simulink model "simulate_gofa_2023"  (R2023a)
settings: Solver=FixedStepAuto  StartTime=0.0  StopTime=100  RelTol=1e-3
undefined symbols (not defined in the file or in its folder): X, Y, Z
libraries: sm_lib x126, nesl_utility x14
(part 3 of 3)

== system simulate_gofa_2023/GOFA robot/link_6 ==
  ReferenceFrame : sm_lib/Frames and Transforms/Reference Frame
  Visual : sm_lib/Body Elements/File Solid  ExtGeomFileName=link_6.stl  UnitType=Custom  ExtGeomFileUnits=m  StepReaderType=HEX  ExportConvexHullGeometry=off  InertiaType=Custom  BasedOnType=DensityFromFile  Density=1000  DensityUnits=kg/m^3  Mass=0  MassUnits=kg  CenterOfMass=[0, 0, 0]  CenterOfMassUnits=m  MomentsOfInertia=[0, 0, 0]  MomentsOfInertiaUnits=kg*m^2  ProductsOfInertia=[0, 0, 0]  ProductsOfInertiaUnits=kg*m^2  GraphicType=FromGeometry  MarkerShape=Sphere  MarkerSize=10  GraphicVisPropType=SimpleVisualProperties  GraphicDiffuseColor=[0.8392157, 0.8352941, 0.7921569000000001]  GraphicOpacity=1  GraphicSpecularColor=[0.5 0.5 0.5 1.0]  GraphicAmbientColor=[0.15 0.15 0.15 1.0]  GraphicEmissiveColor=[0.0 0.0 0.0 1.0]  GraphicShininess=75  DoExposeReferenceFrame=on  SerializedFrames=<Frames/>
  VisualOriginTransform : sm_lib/Frames and Transforms/Rigid Transform  RotationMethod=RotationSequence  FollAlignAxisA=+X  BaseAlignAxisA=+Y  FollAlignAxisB=+Y  BaseAlignAxisB=+Z  RotationStandardAxis=+Z  RotationAngle=0  RotationAngleUnits=deg  RotationArbitraryAxis=[0 0 1]  RotationSequenceAxes=BaseAxes  RotationSequence=XYZ  RotationSequenceAngles=[0, 0, 0]  RotationSequenceAnglesUnits=rad  RotationMatrix=[1 0 0;0 1 0;0 0 1]  Quaternion=[1 0 0 0]  TranslationMethod=Cartesian  TranslationCartesianOffset=[0, 0, 0]  TranslationCartesianOffsetUnits=m  TranslationStandardAxis=+Z  TranslationStandardOffset=0  TranslationStandardOffsetUnits=m  TranslationROffset=0  TranslationROffsetUnits=m  TranslationThetaOffset=0  TranslationThetaOffsetUnits=deg  TranslationZOffset=0  TranslationZOffsetUnits=m
  joint_6_AxisInvTransform : sm_lib/Frames and Transforms/Rigid Transform  RotationMethod=ArbitraryAxis  FollAlignAxisA=+X  BaseAlignAxisA=+Y  FollAlignAxisB=+Y  BaseAlignAxisB=+Z  RotationStandardAxis=+Z  RotationAngle=1.570796326794897  RotationAngleUnits=rad  RotationArbitraryAxis=[-0, 1, 0]  RotationSequenceAxes=FollowerAxes  RotationSequence=XYX  RotationSequenceAngles=[0 0 0]  RotationSequenceAnglesUnits=deg  RotationMatrix=[1 0 0;0 1 0;0 0 1]  Quaternion=[1 0 0 0]  TranslationMethod=Cartesian  TranslationCartesianOffset=[0, 0, 0]  TranslationCartesianOffsetUnits=m  TranslationStandardAxis=+Z  TranslationStandardOffset=0  TranslationStandardOffsetUnits=m  TranslationROffset=0  TranslationROffsetUnits=m  TranslationThetaOffset=0  TranslationThetaOffsetUnits=deg  TranslationZOffset=0  TranslationZOffsetUnits=m
  joint_6_flange_OriginTransform : sm_lib/Frames and Transforms/Rigid Transform  RotationMethod=RotationSequence  FollAlignAxisA=+X  BaseAlignAxisA=+Y  FollAlignAxisB=+Y  BaseAlignAxisB=+Z  RotationStandardAxis=+Z  RotationAngle=0  RotationAngleUnits=deg  RotationArbitraryAxis=[0 0 1]  RotationSequenceAxes=BaseAxes  RotationSequence=XYZ  RotationSequenceAngles=[0, 0, 0]  RotationSequenceAnglesUnits=rad  RotationMatrix=[1 0 0;0 1 0;0 0 1]  Quaternion=[1 0 0 0]  TranslationMethod=Cartesian  TranslationCartesianOffset=[0, 0, 0]  TranslationCartesianOffsetUnits=m  TranslationStandardAxis=+Z  TranslationStandardOffset=0  TranslationStandardOffsetUnits=m  TranslationROffset=0  TranslationROffsetUnits=m  TranslationThetaOffset=0  TranslationThetaOffsetUnits=deg  TranslationZOffset=0  TranslationZOffsetUnits=m
  F : PMIOPort  Side=Left
  F1 : PMIOPort  Port=2  Side=Right
  connections:
  ReferenceFrame/RConn1 -- VisualOriginTransform/LConn1 -- joint_6_AxisInvTransform/LConn1 -- joint_6_flange_OriginTransform/LConn1
  Visual/RConn1 -- VisualOriginTransform/RConn1
  joint_6_AxisInvTransform/RConn1 -- F/RConn1
  joint_6_flange_OriginTransform/RConn1 -- F1/RConn1

== system simulate_gofa_2023/GOFA robot/tool0 ==
  ReferenceFrame : sm_lib/Frames and Transforms/Reference Frame
  F : PMIOPort  Side=Left
  connections:
  ReferenceFrame/RConn1 -- F/RConn1

== matlab function simulate_gofa_2023/GOFA ROBOT KINEMATIC ==
  data: x output; t1 input; y output; t2 input; t3 input; t4 input; t5 input; t6 input; z output; R output
function [x,y,z,R] = fcn(t1,t2,t3,t4,t5,t6)

% Constant params
% d3= 0.15;
% a2 = 0.4318;
% a3 = 0.0203;
% d4 = 0.4318;
% d5 = 0.1;

% end effector position
x = (646333333153388974303668854092654500447200796230458690753650903093*sin((180*t1)/pi))/3291009114642412084309938365114701009965471731267159726697218048000 + (1641179897212867899457543764218157*cos((180*t4)/pi)*((16210310927856405661316834439721*sin((180*t1)/pi))/20282409603651670423947251286016 - (4035888341267763*cos((180*t3)/pi)*((4035888341267763*cos((180*t2)/pi - 90)*sin((180*t1)/pi))/9007199254740992 - sin((180*t2)/pi - 90)*cos((180*t1)/pi)))/9007199254740992 + (4035888341267763*sin((180*t3)/pi)*(cos((180*t2)/pi - 90)*cos((180*t1)/pi) + (4035888341267763*sin((180*t2)/pi - 90)*sin((180*t1)/pi))/9007199254740992))/9007199254740992))/40564819207303340847894502572032000 + (11*cos((180*t3)/pi)*(cos((180*t2)/pi - 90)*cos((180*t1)/pi) + (4035888341267763*sin((180*t2)/pi - 90)*sin((180*t1)/pi))/9007199254740992))/100 + (160146485358502555991456785001454542799219708017911*cos((180*t3)/pi)*((4035888341267763*cos((180*t2)/pi - 90)*sin((180*t1)/pi))/9007199254740992 - sin((180*t2)/pi - 90)*cos((180*t1)/pi)))/365375409332725729550921208179070754913983135744000 - (160146485358502555991456785001454542799219708017911*sin((180*t3)/pi)*(cos((180*t2)/pi - 90)*cos((180*t1)/pi) + (4035888341267763*sin((180*t2)/pi - 90)*sin((180*t1)/pi))/9007199254740992))/365375409332725729550921208179070754913983135744000 + (11*sin((180*t3)/pi)*((4035888341267763*cos((180*t2)/pi - 90)*sin((180*t1)/pi))/9007199254740992 - sin((180*t2)/pi - 90)*cos((180*t1)/pi)))/100 + (2*cos((180*t5)/pi)*(sin((180*t4)/pi)*((16210310927856405661316834439721*sin((180*t1)/pi))/20282409603651670423947251286016 - (4035888341267763*cos((180*t3)/pi)*((4035888341267763*cos((180*t2)/pi - 90)*sin((180*t1)/pi))/9007199254740992 - sin((180*t2)/pi - 90)*cos((180*t1)/pi)))/9007199254740992 + (4035888341267763*sin((180*t3)/pi)*(cos((180*t2)/pi - 90)*cos((180*t1)/pi) + (4035888341267763*sin((180*t2)/pi - 90)*sin((180*t1)/pi))/9007199254740992))/9007199254740992) + cos((180*t4)/pi)*(cos((180*t3)/pi)*(cos((180*t2)/pi - 90)*cos((180*t1)/pi) + (4035888341267763*sin((180*t2)/pi - 90)*sin((180*t1)/pi))/9007199254740992) + sin((180*t3)/pi)*((4035888341267763*cos((180*t2)/pi - 90)*sin((180*t1)/pi))/9007199254740992 - sin((180*t2)/pi - 90)*cos((180*t1)/pi)))))/25 - (1641179897212867899457543764218157*sin((180*t4)/pi)*(cos((180*t3)/pi)*(cos((180*t2)/pi - 90)*cos((180*t1)/pi) + (4035888341267763*sin((180*t2)/pi - 90)*sin((180*t1)/pi))/9007199254740992) + sin((180*t3)/pi)*((4035888341267763*cos((180*t2)/pi - 90)*sin((180*t1)/pi))/9007199254740992 - sin((180*t2)/pi - 90)*cos((180*t1)/pi))))/40564819207303340847894502572032000 - (406646507147255839*sin((180*t5)/pi)*(sin((180*t4)/pi)*((16210310927856405661316834439721*sin((180*t1)/pi))/20282409603651670423947251286016 - (4035888341267763*cos((180*t3)/pi)*((4035888341267763*cos((180*t2)/pi - 90)*sin((180*t1)/pi))/9007199254740992 - sin((180*t2)/pi - 90)*cos((180*t1)/pi)))/9007199254740992 + (4035888341267763*sin((180*t3)/pi)*(cos((180*t2)/pi - 90)*cos((180*t1)/pi) + (4035888341267763*sin((180*t2)/pi - 90)*sin((180*t1)/pi))/9007199254740992))/9007199254740992) + cos((180*t4)/pi)*(cos((180*t3)/pi)*(cos((180*t2)/pi - 90)*cos((180*t1)/pi) + (4035888341267763*sin((180*t2)/pi - 90)*sin((180*t1)/pi))/9007199254740992) + sin((180*t3)/pi)*((4035888341267763*cos((180*t2)/pi - 90)*sin((180*t1)/pi))/9007199254740992 - sin((180*t2)/pi - 90)*cos((180*t1)/pi)))))/4503599627370496000 + (11*cos((180*t2)/pi - 90)*cos((180*t1)/pi))/25 + (406646507147255839*cos((180*t5)/pi)*((65423004882061081215650621571388430732944014123*sin((180*t1)/pi))/182687704666362864775460604089535377456991567872 - (4035888341267763*cos((180*t4)/pi)*((16210310927856405661316834439721*sin((180*t1)/pi))/20282409603651670423947251286016 - (4035888341267763*cos((180*t3)/pi)*((4035888341267763*cos((180*t2)/pi - 90)*sin((180*t1)/pi))/9007199254740992 - sin((180*t2)/pi - 90)*cos((180*t1)/pi)))/9007199254740992 + (4035888341267763*sin((180*t3)/pi)*(cos((180*t2)/pi - 90)*cos((180*t1)/pi) + (4035888341267763*sin((180*t2)/pi - 90)*sin((180*t1)/pi))/9007199254740992))/9007199254740992))/9007199254740992 + (16210310927856405661316834439721*cos((180*t3)/pi)*((4035888341267763*cos((180*t2)/pi - 90)*sin((180*t1)/pi))/9007199254740992 - sin((180*t2)/pi - 90)*cos((180*t1)/pi)))/20282409603651670423947251286016 - (16210310927856405661316834439721*sin((180*t3)/pi)*(cos((180*t2)/pi - 90)*cos((180*t1)/pi) + (4035888341267763*sin((180*t2)/pi - 90)*sin((180*t1)/pi))/9007199254740992))/20282409603651670423947251286016 + (4035888341267763*sin((180*t4)/pi)*(cos((180*t3)/pi)*(cos((180*t2)/pi - 90)*cos((180*t1)/pi) + (4035888341267763*sin((180*t2)/pi - 90)*sin((180*t1)/pi))/9007199254740992) + sin((180*t3)/pi)*((4035888341267763*cos((180*t2)/pi - 90)*sin((180*t1)/pi))/9007199254740992 - sin((180*t2)/pi - 90)*cos((180*t1)/pi))))/9007199254740992))/4503599627370496000 + (44394771753945393*sin((180*t2)/pi - 90)*sin((180*t1)/pi))/225179981368524800 + (2*sin((180*t5)/pi)*((65423004882061081215650621571388430732944014123*sin((180*t1)/pi))/182687704666362864775460604089535377456991567872 - (4035888341267763*cos((180*t4)/pi)*((16210310927856405661316834439721*sin((180*t1)/pi))/20282409603651670423947251286016 - (4035888341267763*cos((180*t3)/pi)*((4035888341267763*cos((180*t2)/pi - 90)*sin((180*t1)/pi))/9007199254740992 - sin((180*t2)/pi - 90)*cos((180*t1)/pi)))/9007199254740992 + (4035888341267763*sin((180*t3)/pi)*(cos((180*t2)/pi - 90)*cos((180*t1)/pi) + (4035888341267763*sin((180*t2)/pi - 90)*sin((180*t1)/pi))/9007199254740992))/9007199254740992))/9007199254740992 + (16210310927856405661316834439721*cos((180*t3)/pi)*((4035888341267763*cos((180*t2)/pi - 90)*sin((180*t1)/pi))/9007199254740992 - sin((180*t2)/pi - 90)*cos((180*t1)/pi)))/20282409603651670423947251286016 - (16210310927856405661316834439721*sin((180*t3)/pi)*(cos((180*t2)/pi - 90)*cos((180*t1)/pi) + (4035888341267763*sin((180*t2)/pi - 90)*sin((180*t1)/pi))/9007199254740992))/20282409603651670423947251286016 + (4035888341267763*sin((180*t4)/pi)*(cos((180*t3)/pi)*(cos((180*t2)/pi - 90)*cos((180*t1)/pi) + (4035888341267763*sin((180*t2)/pi - 90)*sin((180*t1)/pi))/9007199254740992) + sin((180*t3)/pi)*((4035888341267763*cos((180*t2)/pi - 90)*sin((180*t1)/pi))/9007199254740992 - sin((180*t2)/pi - 90)*cos((180*t1)/pi))))/9007199254740992))/25;

y = (1641179897212867899457543764218157*cos((180*t4)/pi)*((4035888341267763*cos((180*t3)/pi)*((4035888341267763*cos((180*t2)/pi - 90)*cos((180*t1)/pi))/9007199254740992 + sin((180*t2)/pi - 90)*sin((180*t1)/pi)))/9007199254740992 - (16210310927856405661316834439721*cos((180*t1)/pi))/20282409603651670423947251286016 + (4035888341267763*sin((180*t3)/pi)*(cos((180*t2)/pi - 90)*sin((180*t1)/pi) - (4035888341267763*sin((180*t2)/pi - 90)*cos((180*t1)/pi))/9007199254740992))/9007199254740992))/40564819207303340847894502572032000 - (646333333153388974303668854092654500447200796230458690753650903093*cos((180*t1)/pi))/3291009114642412084309938365114701009965471731267159726697218048000 + (11*cos((180*t3)/pi)*(cos((180*t2)/pi - 90)*sin((180*t1)/pi) - (4035888341267763*sin((180*t2)/pi - 90)*cos((180*t1)/pi))/9007199254740992))/100 - (160146485358502555991456785001454542799219708017911*cos((180*t3)/pi)*((4035888341267763*cos((180*t2)/pi - 90)*cos((180*t1)/pi))/9007199254740992 + sin((180*t2)/pi - 90)*sin((180*t1)/pi)))/365375409332725729550921208179070754913983135744000 + (2*cos((180*t5)/pi)*(sin((180*t4)/pi)*((4035888341267763*cos((180*t3)/pi)*((4035888341267763*cos((180*t2)/pi - 90)*cos((180*t1)/pi))/9007199254740992 + sin((180*t2)/pi - 90)*sin((180*t1)/pi)))/9007199254740992 - (16210310927856405661316834439721*cos((180*t1)/pi))/20282409603651670423947251286016 + (4035888341267763*sin((180*t3)/pi)*(cos((180*t2)/pi - 90)*sin((180*t1)/pi) - (4035888341267763*sin((180*t2)/pi - 90)*cos((180*t1)/pi))/9007199254740992))/9007199254740992) + cos((180*t4)/pi)*(cos((180*t3)/pi)*(cos((180*t2)/pi - 90)*sin((180*t1)/pi) - (4035888341267763*sin((180*t2)/pi - 90)*cos((180*t1)/pi))/9007199254740992) - sin((180*t3)/pi)*((4035888341267763*cos((180*t2)/pi - 90)*cos((180*t1)/pi))/9007199254740992 + sin((180*t2)/pi - 90)*sin((180*t1)/pi)))))/25 - (160146485358502555991456785001454542799219708017911*sin((180*t3)/pi)*(cos((180*t2)/pi - 90)*sin((180*t1)/pi) - (4035888341267763*sin((180*t2)/pi - 90)*cos((180*t1)/pi))/9007199254740992))/365375409332725729550921208179070754913983135744000 - (11*sin((180*t3)/pi)*((4035888341267763*cos((180*t2)/pi - 90)*cos((180*t1)/pi))/9007199254740992 + sin((180*t2)/pi - 90)*sin((180*t1)/pi)))/100 - (406646507147255839*sin((180*t5)/pi)*(sin((180*t4)/pi)*((4035888341267763*cos((180*t3)/pi)*((4035888341267763*cos((180*t2)/pi - 90)*cos((180*t1)/pi))/9007199254740992 + sin((180*t2)/pi - 90)*sin((180*t1)/pi)))/9007199254740992 - (16210310927856405661316834439721*cos((180*t1)/pi))/20282409603651670423947251286016 + (4035888341267763*sin((180*t3)/pi)*(cos((180*t2)/pi - 90)*sin((180*t1)/pi) - (4035888341267763*sin((180*t2)/pi - 90)*cos((180*t1)/pi))/9007199254740992))/9007199254740992) + cos((180*t4)/pi)*(cos((180*t3)/pi)*(cos((180*t2)/pi - 90)*sin((180*t1)/pi) - (4035888341267763*sin((180*t2)/pi - 90)*cos((180*t1)/pi))/9007199254740992) - sin((180*t3)/pi)*((4035888341267763*cos((180*t2)/pi - 90)*cos((180*t1)/pi))/9007199254740992 + sin((180*t2)/pi - 90)*sin((180*t1)/pi)))))/4503599627370496000 - (1641179897212867899457543764218157*sin((180*t4)/pi)*(cos((180*t3)/pi)*(cos((180*t2)/pi - 90)*sin((180*t1)/pi) - (4035888341267763*sin((180*t2)/pi - 90)*cos((180*t1)/pi))/9007199254740992) - sin((180*t3)/pi)*((4035888341267763*cos((180*t2)/pi - 90)*cos((180*t1)/pi))/9007199254740992 + sin((180*t2)/pi - 90)*sin((180*t1)/pi))))/40564819207303340847894502572032000 - (406646507147255839*cos((180*t5)/pi)*((65423004882061081215650621571388430732944014123*cos((180*t1)/pi))/182687704666362864775460604089535377456991567872 + (4035888341267763*cos((180*t4)/pi)*((4035888341267763*cos((180*t3)/pi)*((4035888341267763*cos((180*t2)/pi - 90)*cos((180*t1)/pi))/9007199254740992 + sin((180*t2)/pi - 90)*sin((180*t1)/pi)))/9007199254740992 - (16210310927856405661316834439721*cos((180*t1)/pi))/20282409603651670423947251286016 + (4035888341267763*sin((180*t3)/pi)*(cos((180*t2)/pi - 90)*sin((180*t1)/pi) - (4035888341267763*sin((180*t2)/pi - 90)*cos((180*t1)/pi))/9007199254740992))/9007199254740992))/9007199254740992 + (16210310927856405661316834439721*cos((180*t3)/pi)*((4035888341267763*cos((180*t2)/pi - 90)*cos((180*t1)/pi))/9007199254740992 + sin((180*t2)/pi - 90)*sin((180*t1)/pi)))/20282409603651670423947251286016 + (16210310927856405661316834439721*sin((180*t3)/pi)*(cos((180*t2)/pi - 90)*sin((180*t1)/pi) - (4035888341267763*sin((180*t2)/pi - 90)*cos((180*t1)/pi))/9007199254740992))/20282409603651670423947251286016 - (4035888341267763*sin((180*t4)/pi)*(cos((180*t3)/pi)*(cos((180*t2)/pi - 90)*sin((180*t1)/pi) - (4035888341267763*sin((180*t2)/pi - 90)*cos((180*t1)/pi))/9007199254740992) - sin((180*t3)/pi)*((4035888341267763*cos((180*t2)/pi - 90)*cos((180*t1)/pi))/9007199254740992 + sin((180*t2)/pi - 90)*sin((180*t1)/pi))))/9007199254740992))/4503599627370496000 - (2*sin((180*t5)/pi)*((65423004882061081215650621571388430732944014123*cos((180*t1)/pi))/182687704666362864775460604089535377456991567872 + (4035888341267763*cos((180*t4)/pi)*((4035888341267763*cos((180*t3)/pi)*((4035888341267763*cos((180*t2)/pi - 90)*cos((180*t1)/pi))/9007199254740992 + sin((180*t2)/pi - 90)*sin((180*t1)/pi)))/9007199254740992 - (16210310927856405661316834439721*cos((180*t1)/pi))/20282409603651670423947251286016 + (4035888341267763*sin((180*t3)/pi)*(cos((180*t2)/pi - 90)*sin((180*t1)/pi) - (4035888341267763*sin((180*t2)/pi - 90)*cos((180*t1)/pi))/9007199254740992))/9007199254740992))/9007199254740992 + (16210310927856405661316834439721*cos((180*t3)/pi)*((4035888341267763*cos((180*t2)/pi - 90)*cos((180*t1)/pi))/9007199254740992 + sin((180*t2)/pi - 90)*sin((180*t1)/pi)))/20282409603651670423947251286016 + (16210310927856405661316834439721*sin((180*t3)/pi)*(cos((180*t2)/pi - 90)*sin((180*t1)/pi) - (4035888341267763*sin((180*t2)/pi - 90)*cos((180*t1)/pi))/9007199254740992))/20282409603651670423947251286016 - (4035888341267763*sin((180*t4)/pi)*(cos((180*t3)/pi)*(cos((180*t2)/pi - 90)*sin((180*t1)/pi) - (4035888341267763*sin((180*t2)/pi - 90)*cos((180*t1)/pi))/9007199254740992) - sin((180*t3)/pi)*((4035888341267763*cos((180*t2)/pi - 90)*cos((180*t1)/pi))/9007199254740992 + sin((180*t2)/pi - 90)*sin((180*t1)/pi))))/9007199254740992))/25 + (11*cos((180*t2)/pi - 90)*sin((180*t1)/pi))/25 - (44394771753945393*sin((180*t2)/pi - 90)*cos((180*t1)/pi))/225179981368524800;

z = (6607723493088169202780712778710231504027345426423*sin((180*t2)/pi + (180*t3)/pi - 90)*sin((180*t4)/pi))/182687704666362864775460604089535377456991567872000 - (644782266365784279295696367608494311447688133775286220162272389429*cos((180*t2)/pi + (180*t3)/pi - 90))/1645504557321206042154969182557350504982735865633579863348609024000 - (44288233451681329*sin((180*t2)/pi + (180*t3)/pi - 90))/450359962737049600 - cos((180*t5)/pi)*((26540192218155861146320042886836656302738191977718887318238341941*cos((180*t2)/pi + (180*t3)/pi - 90))/411376139330301510538742295639337626245683966408394965837152256000 + (406646507147255839*cos((180*t4)/pi)*((65580384287964744588230398513542208987583003691*cos((180*t2)/pi + (180*t3)/pi - 90))/365375409332725729550921208179070754913983135744 + 65580384287964744588230398513542208987583003691/365375409332725729550921208179070754913983135744))/4503599627370496000 + (6607723493088169202780712778710231504027345426423*sin((180*t2)/pi + (180*t3)/pi - 90)*sin((180*t4)/pi))/182687704666362864775460604089535377456991567872000 - 26668034208075640036217710933510508340280645669893133127658301749/1645504557321206042154969182557350504982735865633579863348609024000) - sin((180*t5)/pi)*((406646507147255839*sin((180*t4)/pi)*((16249305912998692073837066972457*cos((180*t2)/pi + (180*t3)/pi - 90))/40564819207303340847894502572032 + 16249305912998692073837066972457/40564819207303340847894502572032))/4503599627370496000 - (1637241403713496971793000278411821*sin((180*t2)/pi + (180*t3)/pi - 90)*cos((180*t4)/pi))/20282409603651670423947251286016000) - (44288233451681329*sin((180*t2)/pi - 90))/112589990684262400 + cos((180*t5)/pi)*((2*sin((180*t4)/pi)*((16249305912998692073837066972457*cos((180*t2)/pi + (180*t3)/pi - 90))/40564819207303340847894502572032 + 16249305912998692073837066972457/40564819207303340847894502572032))/25 - (4026203041061939*sin((180*t2)/pi + (180*t3)/pi - 90)*cos((180*t4)/pi))/56294995342131200) - sin((180*t5)/pi)*((65266003154295042533483952795954524799922879019*cos((180*t2)/pi + (180*t3)/pi - 90))/1141798154164767904846628775559596109106197299200 + (2*cos((180*t4)/pi)*((65580384287964744588230398513542208987583003691*cos((180*t2)/pi + (180*t3)/pi - 90))/365375409332725729550921208179070754913983135744 + 65580384287964744588230398513542208987583003691/365375409332725729550921208179070754913983135744))/25 + (16249305912998692073837066972457*sin((180*t2)/pi + (180*t3)/pi - 90)*sin((180*t4)/pi))/507060240091291760598681282150400 - 65580384287964744588230398513542208987583003691/4567192616659071619386515102238384436424789196800) + cos((180*t4)/pi)*((26668034208075640036217710933510508340280645669893133127658301749*cos((180*t2)/pi + (180*t3)/pi - 90))/1645504557321206042154969182557350504982735865633579863348609024000 + 26668034208075640036217710933510508340280645669893133127658301749/1645504557321206042154969182557350504982735865633579863348609024000) + 2392122961896179351406805570435440567063495989399766582953892685621/6582018229284824168619876730229402019930943462534319453394436096000;

r_matrix = zeros(3,3);

r_matrix(1,1) = - cos((pi*((180*t3)/pi + (180*t4)/pi))/180)*cos(t6) - sin((pi*((180*t3)/pi + (180*t4)/pi))/180)*cos(t5)*sin(t6);
r_matrix(1,2) = -sin((pi*((180*t3)/pi + (180*t4)/pi))/180)*sin(t5);
r_matrix(1,3) = sin((pi*((180*t3)/pi + (180*t4)/pi))/180)*cos(t5)*cos(t6) - cos((pi*((180*t3)/pi + (180*t4)/pi))/180)*sin(t6);


r_matrix(2,1) = cos((pi*((180*t1)/pi - (180*t2)/pi))/180)*sin((pi*((180*t3)/pi + (180*t4)/pi))/180)*cos(t6) - sin(t6)*(sin((pi*((180*t1)/pi - (180*t2)/pi))/180)*sin(t5) + cos((pi*((180*t1)/pi - (180*t2)/pi))/180)*cos((pi*((180*t3)/pi + (180*t4)/pi))/180)*cos(t5));
r_matrix(2,2) = sin((pi*((180*t1)/pi - (180*t2)/pi))/180)*cos(t5) - cos((pi*((180*t1)/pi - (180*t2)/pi))/180)*cos((pi*((180*t3)/pi + (180*t4)/pi))/180)*sin(t5);
r_matrix(2,3) = cos(t6)*(sin((pi*((180*t1)/pi - (180*t2)/pi))/180)*sin(t5) + cos((pi*((180*t1)/pi - (180*t2)/pi))/180)*cos((pi*((180*t3)/pi + (180*t4)/pi))/180)*cos(t5)) + cos((pi*((180*t1)/pi - (180*t2)/pi))/180)*sin((pi*((180*t3)/pi + (180*t4)/pi))/180)*sin(t6);

r_matrix(3,1) = - sin(t6)*(cos((pi*((180*t1)/pi - (180*t2)/pi))/180)*sin(t5) - cos((pi*((180*t3)/pi + (180*t4)/pi))/180)*sin((pi*((180*t1)/pi - (180*t2)/pi))/180)*cos(t5)) - sin((pi*((180*t1)/pi - (180*t2)/pi))/180)*sin((pi*((180*t3)/pi + (180*t4)/pi))/180)*cos(t6);
r_matrix(3,2) = cos((pi*((180*t1)/pi - (180*t2)/pi))/180)*cos(t5) + cos((pi*((180*t3)/pi + (180*t4)/pi))/180)*sin((pi*((180*t1)/pi - (180*t2)/pi))/180)*sin(t5);
r_matrix(3,3) = cos(t6)*(cos((pi*((180*t1)/pi - (180*t2)/pi))/180)*sin(t5) - cos((pi*((180*t3)/pi + (180*t4)/pi))/180)*sin((pi*((180*t1)/pi - (180*t2)/pi))/180)*cos(t5)) - sin((pi*((180*t1)/pi - (180*t2)/pi))/180)*sin((pi*((180*t3)/pi + (180*t4)/pi))/180)*sin(t6);
R = r_matrix;

== matlab function simulate_gofa_2023/Inverse Jacobian ==
  settings: updateMethod=DISCRETE
  data: dx input; dy input; dz input; d_alpha input; d_beta input; d_gamma input; output_joint_value output; output_djoint_value output; joint_value input; det_J output
function [output_joint_value,output_djoint_value,det_J] = ...
    fcn(dx,dy,dz,d_alpha,d_beta,d_gamma, joint_value)

% ===== Cấu hình nhanh =====
treatAsRate = true;   % true: dx.. = tốc độ (twist); false: dx.. = bước dịch
dt           = 0.01;  % dùng khi treatAsRate==true
useDLS       = true;  % dùng damped least squares cho ổn định
lambda       = 0.001;  % hệ số damping

assert(isnumeric(joint_value) && isvector(joint_value) && numel(joint_value)==6);
q = reshape(joint_value,6,1);
t1=q(1); t2=q(2); t3=q(3); t4=q(4); t5=q(5); t6=q(6);

% ===== Jacobian GOFA (bạn đã tính) =====
J = zeros(6,6);

J(1,1) = 0;
J(1,2) = 0;
J(1,3) = (111*cos(t3))/250 + (11*cos(t3)*cos(t4))/100 - (11*sin(t3)*sin(t4))/100 + (2*cos(t3)*sin(t4)*sin(t6))/25 + (2*cos(t4)*sin(t3)*sin(t6))/25 + (101*cos(t3)*cos(t6)*sin(t4))/1000 + (101*cos(t4)*cos(t6)*sin(t3))/1000 + (2*cos(t3)*cos(t4)*cos(t5)*cos(t6))/25 - (101*cos(t3)*cos(t4)*cos(t5)*sin(t6))/1000 - (2*cos(t5)*cos(t6)*sin(t3)*sin(t4))/25 + (101*cos(t5)*sin(t3)*sin(t4)*sin(t6))/1000;
J(1,4) = (11*cos(t3)*cos(t4))/100 - (11*sin(t3)*sin(t4))/100 + (2*cos(t3)*sin(t4)*sin(t6))/25 + (2*cos(t4)*sin(t3)*sin(t6))/25 + (101*cos(t3)*cos(t6)*sin(t4))/1000 + (101*cos(t4)*cos(t6)*sin(t3))/1000 + (2*cos(t3)*cos(t4)*cos(t5)*cos(t6))/25 - (101*cos(t3)*cos(t4)*cos(t5)*sin(t6))/1000 - (2*cos(t5)*cos(t6)*sin(t3)*sin(t4))/25 + (101*cos(t5)*sin(t3)*sin(t4)*sin(t6))/1000;
J(1,5) = -(sin(t3 + t4)*sin(t5)*(80*cos(t6) - 101*sin(t6)))/1000;
J(1,6) = (101*cos(t3 + t4)*sin(t6))/1000 - (2*cos(t3 + t4)*cos(t6))/25 - (101*sin(t3 + t4)*cos(t5)*cos(t6))/1000 - (2*sin(t3 + t4)*cos(t5)*sin(t6))/25;

J(2,1) = (2*cos(t1 - t2)*cos(t6)*sin(t5))/25 - (47*sin(t1)*sin(t2))/100 - (111*sin(t1 - t2)*cos(t3))/250 - (101*sin(t1 - t2)*sin(t3 + t4)*cos(t6))/1000 - (2*sin(t1 - t2)*sin(t3 + t4)*sin(t6))/25 - (11*sin(t1 - t2)*cos(t3)*cos(t4))/100 - (47*cos(t1)*cos(t2))/100 - (101*cos(t1 - t2)*sin(t5)*sin(t6))/1000 + (11*sin(t1 - t2)*sin(t3)*sin(t4))/100 - (2*sin(t1 - t2)*cos(t3 + t4)*cos(t5)*cos(t6))/25 + (101*sin(t1 - t2)*cos(t3 + t4)*cos(t5)*sin(t6))/1000;
J(2,2) = (47*cos(t1)*cos(t2))/100 + (47*sin(t1)*sin(t2))/100 + (111*sin(t1 - t2)*cos(t3))/250 + (101*sin(t1 - t2)*sin(t3 + t4)*cos(t6))/1000 + (2*sin(t1 - t2)*sin(t3 + t4)*sin(t6))/25 + (11*sin(t1 - t2)*cos(t3)*cos(t4))/100 - (2*cos(t1 - t2)*cos(t6)*sin(t5))/25 + (101*cos(t1 - t2)*sin(t5)*sin(t6))/1000 - (11*sin(t1 - t2)*sin(t3)*sin(t4))/100 + (2*sin(t1 - t2)*cos(t3 + t4)*cos(t5)*cos(t6))/25 - (101*sin(t1 - t2)*cos(t3 + t4)*cos(t5)*sin(t6))/1000;
J(2,3) = -(cos(t1 - t2)*(444*sin(t3) + 110*cos(t3)*sin(t4) + 110*cos(t4)*sin(t3) + 101*cos(t6)*sin(t3)*sin(t4) + 80*sin(t3)*sin(t4)*sin(t6) - 101*cos(t3)*cos(t4)*cos(t6) - 80*cos(t3)*cos(t4)*sin(t6) + 80*cos(t3)*cos(t5)*cos(t6)*sin(t4) + 80*cos(t4)*cos(t5)*cos(t6)*sin(t3) - 101*cos(t3)*cos(t5)*sin(t4)*sin(t6) - 101*cos(t4)*cos(t5)*sin(t3)*sin(t6)))/1000;
J(2,4) = -(cos(t1 - t2)*(110*cos(t3)*sin(t4) + 110*cos(t4)*sin(t3) + 101*cos(t6)*sin(t3)*sin(t4) + 80*sin(t3)*sin(t4)*sin(t6) - 101*cos(t3)*cos(t4)*cos(t6) - 80*cos(t3)*cos(t4)*sin(t6) + 80*cos(t3)*cos(t5)*cos(t6)*sin(t4) + 80*cos(t4)*cos(t5)*cos(t6)*sin(t3) - 101*cos(t3)*cos(t5)*sin(t4)*sin(t6) - 101*cos(t4)*cos(t5)*sin(t3)*sin(t6)))/1000;
J(2,5) = ((sin(t1 - t2)*cos(t5) - cos(t1 - t2)*cos(t3 + t4)*sin(t5))*(80*cos(t6) - 101*sin(t6)))/1000;
J(2,6) = (2*cos(t1 - t2)*sin(t3 + t4)*cos(t6))/25 - (2*sin(t6)*(sin(t1 - t2)*sin(t5) + cos(t1 - t2)*cos(t3 + t4)*cos(t5)))/25 - (101*cos(t1 - t2)*sin(t3 + t4)*sin(t6))/1000 - (101*cos(t6)*(sin(t1 - t2)*sin(t5) + cos(t1 - t2)*cos(t3 + t4)*cos(t5)))/1000;

J(3,1) = (47*cos(t2)*sin(t1))/100 - (47*cos(t1)*sin(t2))/100 - (111*cos(t1 - t2)*cos(t3))/250 - (2*cos(t1 - t2)*sin(t3 + t4)*sin(t6))/25 - (11*cos(t1 - t2)*cos(t3)*cos(t4))/100 + (11*cos(t1 - t2)*sin(t3)*sin(t4))/100 - (2*sin(t1 - t2)*cos(t6)*sin(t5))/25 + (101*sin(t1 - t2)*sin(t5)*sin(t6))/1000 - (101*cos(t1 - t2)*sin(t3 + t4)*cos(t6))/1000 - (2*cos(t1 - t2)*cos(t3 + t4)*cos(t5)*cos(t6))/25 + (101*cos(t1 - t2)*cos(t3 + t4)*cos(t5)*sin(t6))/1000;
J(3,2) = (47*cos(t1)*sin(t2))/100 - (47*cos(t2)*sin(t1))/100 + (111*cos(t1 - t2)*cos(t3))/250 + (2*cos(t1 - t2)*sin(t3 + t4)*sin(t6))/25 + (11*cos(t1 - t2)*cos(t3)*cos(t4))/100 - (11*cos(t1 - t2)*sin(t3)*sin(t4))/100 + (2*sin(t1 - t2)*cos(t6)*sin(t5))/25 - (101*sin(t1 - t2)*sin(t5)*sin(t6))/1000 + (101*cos(t1 - t2)*sin(t3 + t4)*cos(t6))/1000 + (2*cos(t1 - t2)*cos(t3 + t4)*cos(t5)*cos(t6))/25 - (101*cos(t1 - t2)*cos(t3 + t4)*cos(t5)*sin(t6))/1000; 
J(3,3) = (sin(t1 - t2)*(444*sin(t3) + 110*cos(t3)*sin(t4) + 110*cos(t4)*sin(t3) + 101*cos(t6)*sin(t3)*sin(t4) + 80*sin(t3)*sin(t4)*sin(t6) - 101*cos(t3)*cos(t4)*cos(t6) - 80*cos(t3)*cos(t4)*sin(t6) + 80*cos(t3)*cos(t5)*cos(t6)*sin(t4) + 80*cos(t4)*cos(t5)*cos(t6)*sin(t3) - 101*cos(t3)*cos(t5)*sin(t4)*sin(t6) - 101*cos(t4)*cos(t5)*sin(t3)*sin(t6)))/1000;
J(3,4) = (sin(t1 - t2)*(110*cos(t3)*sin(t4) + 110*cos(t4)*sin(t3) + 101*cos(t6)*sin(t3)*sin(t4) + 80*sin(t3)*sin(t4)*sin(t6) - 101*cos(t3)*cos(t4)*cos(t6) - 80*cos(t3)*cos(t4)*sin(t6) + 80*cos(t3)*cos(t5)*cos(t6)*sin(t4) + 80*cos(t4)*cos(t5)*cos(t6)*sin(t3) - 101*cos(t3)*cos(t5)*sin(t4)*sin(t6) - 101*cos(t4)*cos(t5)*sin(t3)*sin(t6)))/1000; 
J(3,5) = ((cos(t1 - t2)*cos(t5) + sin(t1 - t2)*cos(t3 + t4)*sin(t5))*(80*cos(t6) - 101*sin(t6)))/1000;
J(3,6) = (101*sin(t1 - t2)*sin(t3 + t4)*sin(t6))/1000 - (2*sin(t6)*(cos(t1 - t2)*sin(t5) - sin(t1 - t2)*cos(t3 + t4)*cos(t5)))/25 - (2*sin(t1 - t2)*sin(t3 + t4)*cos(t6))/25 - (101*cos(t6)*(cos(t1 - t2)*sin(t5) - sin(t1 - t2)*cos(t3 + t4)*cos(t5)))/1000;

J(4,1) = 0;
J(4,2) = 0;
J(4,3) = sin(t3);
J(4,4) = sin(t3 + t4);
J(4,5) = sin(t3 + t4)*cos(t5);
J(4,6) = sin(t3 + t4)*cos(t5)*cos(t6) - cos(t3 + t4)*sin(t6);

J(5,1) = sin((pi*((180*t1)/pi - 180))/180);
J(5,2) = cos(t1 - t2);
J(5,3) = cos(t1 - t2)*cos(t3);
J(5,4) = cos(t1 - t2 + t3 + t4)/2 + cos(t2 - t1 + t3 + t4)/2;
J(5,5) = cos(t2)*sin(t1)*sin(t5) - cos(t1)*sin(t2)*sin(t5) + cos(t1)*cos(t2)*cos(t3)*cos(t4)*cos(t5) - cos(t1)*cos(t2)*cos(t5)*sin(t3)*sin(t4) + cos(t3)*cos(t4)*cos(t5)*sin(t1)*sin(t2) - cos(t5)*sin(t1)*sin(t2)*sin(t3)*sin(t4);
J(5,6) = cos(t2)*cos(t6)*sin(t1)*sin(t5) - cos(t1)*cos(t6)*sin(t2)*sin(t5) + cos(t1)*cos(t2)*cos(t3)*sin(t4)*sin(t6) + cos(t1)*cos(t2)*cos(t4)*sin(t3)*sin(t6) + cos(t3)*sin(t1)*sin(t2)*sin(t4)*sin(t6) + cos(t4)*sin(t1)*sin(t2)*sin(t3)*sin(t6) + cos(t1)*cos(t2)*cos(t3)*cos(t4)*cos(t5)*cos(t6) - cos(t1)*cos(t2)*cos(t5)*cos(t6)*sin(t3)*sin(t4) + cos(t3)*cos(t4)*cos(t5)*cos(t6)*sin(t1)*sin(t2) - cos(t5)*cos(t6)*sin(t1)*sin(t2)*sin(t3)*sin(t4);

J(6,1) = cos((pi*((180*t1)/pi - 180))/180);
J(6,2) = -sin(t1 - t2);
J(6,3) = -sin(t1 - t2)*cos(t3);
J(6,4) = sin(t2 - t1 + t3 + t4)/2 - sin(t1 - t2 + t3 + t4)/2;
J(6,5) = sin(t1)*sin(t2)*sin(t5) + cos(t1)*cos(t2)*sin(t5) + cos(t1)*cos(t3)*cos(t4)*cos(t5)*sin(t2) - cos(t2)*cos(t3)*cos(t4)*cos(t5)*sin(t1) - cos(t1)*cos(t5)*sin(t2)*sin(t3)*sin(t4) + cos(t2)*cos(t5)*sin(t1)*sin(t3)*sin(t4);
J(6,6) = cos(t1)*cos(t2)*cos(t6)*sin(t5) + cos(t6)*sin(t1)*sin(t2)*sin(t5) + cos(t1)*cos(t3)*sin(t2)*sin(t4)*sin(t6) + cos(t1)*cos(t4)*sin(t2)*sin(t3)*sin(t6) - cos(t2)*cos(t3)*sin(t1)*sin(t4)*sin(t6) - cos(t2)*cos(t4)*sin(t1)*sin(t3)*sin(t6) + cos(t1)*cos(t3)*cos(t4)*cos(t5)*cos(t6)*sin(t2) - cos(t2)*cos(t3)*cos(t4)*cos(t5)*cos(t6)*sin(t1) - cos(t1)*cos(t5)*cos(t6)*sin(t2)*sin(t3)*sin(t4) + cos(t2)*cos(t5)*cos(t6)*sin(t1)*sin(t3)*sin(t4);

% ===== Giải nghịch Jacobian =====
d_ef = [dx; dy; dz; d_alpha; d_beta; d_gamma];  % 6x1

if useDLS
    % Damped least-squares: ổn định gần kỳ dị
    d_joint = (J.'*J + (lambda^2)*eye(6)) \ (J.'*d_ef);
else
    % Nghịch đảo trực tiếp
    d_joint = J \ d_ef;
end

% ===== Xuất kết quả =====
output_djoint_value = d_joint;      % dq (rad/s)
if treatAsRate
    output_joint_value = q + dt * d_joint;    % cập nhật theo vận tốc
else
    output_joint_value = q + d_joint;         % cập nhật theo bước dịch
end

det_J = det(J);
